simulink model "modele_source"  (R2024b)
settings: Solver=FixedStepDiscrete  StartTime=0.0  StopTime=(Nsim-1)*Tb  FixedStep=Tb  RelTol=1e-3
undefined symbols (not defined in the file or in its folder): graine, p1, Tb
settings Model: Creator=youka  LastModifiedBy=youka

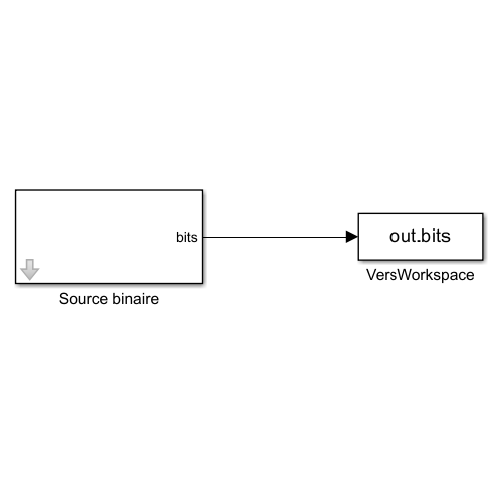
[thumbnail: Simulink's stored preview of the top-level diagram]
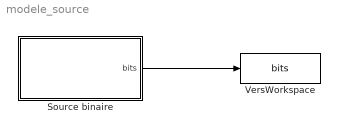
== system modele_source ==
  Source binaire : Subsystem  mask(Source binaire){p1_m=p1, Tb_m=Tb, graine_m=graine}
      mask prompts: p1_m "Probabilité d'émettre un 1 (p1)"; Tb_m "Durée d'un bit Tb (s)"; graine_m "Graine (Seed)"
      mask help: Source binaire sans mémoire : P(1) = p1, un bit toutes les Tb secondes.
  VersWorkspace : ToWorkspace  VariableName=bits  SampleTime=-1
  wires:
  Source binaire/1(bits) -> VersWorkspace/1

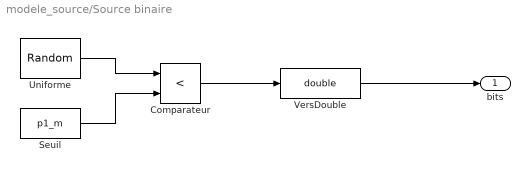
== system modele_source/Source binaire ==
  Comparateur : RelationalOperator  Operator=<  OutDataTypeStr=boolean  RndMeth=Simplest  InputSameDT=off
  Seuil : Constant  Value=p1_m  SampleTime=Tb_m
  Uniforme : UniformRandomNumber  Minimum=0  Seed=graine_m  SampleTime=Tb_m
  VersDouble : DataTypeConversion  OutDataTypeStr=double  SaturateOnIntegerOverflow=off  RndMeth=Floor
  bits : Outport
  wires:
  Uniforme/1 -> Comparateur/1
  Seuil/1 -> Comparateur/2
  Comparateur/1 -> VersDouble/1
  VersDouble/1 -> bits/1
